simulink model "lab3_buck_closed_loop"  (R2025b)
settings: Solver=VariableStepAuto  StartTime=0.0  StopTime=2  RelTol=1e-3
settings Model: Creator=Fer Alexandru  LastModifiedBy=Fer Alexandru

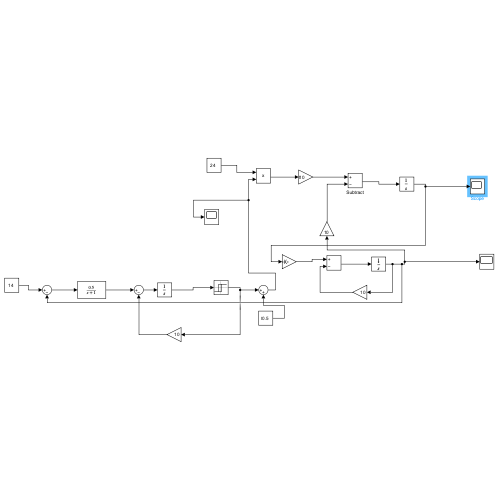
[thumbnail: Simulink's stored preview of the top-level diagram]
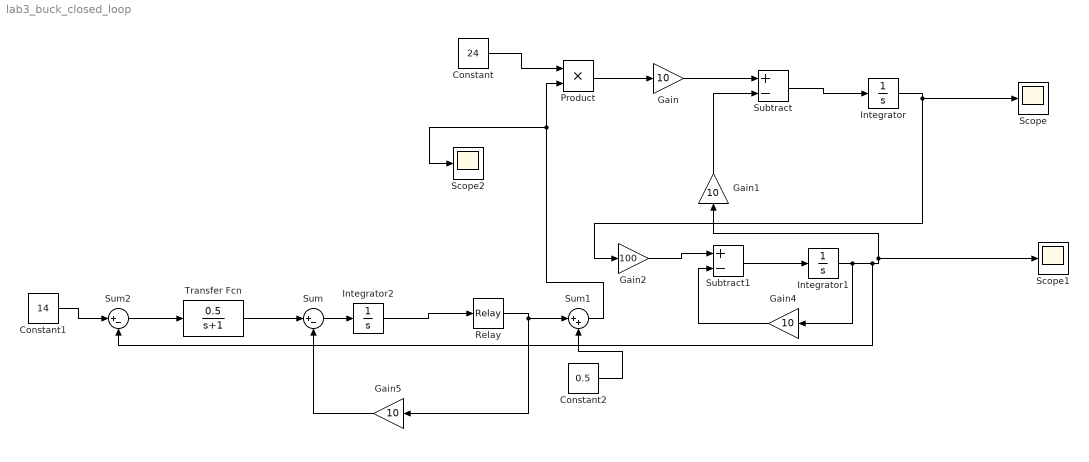
== system lab3_buck_closed_loop ==
  Constant : Constant  Value=24
  Constant1 : Constant  Value=14
  Constant2 : Constant  Value=0.5
  Gain{,1,4..5} (4 alike) : Gain  Gain=10
  Gain2 : Gain  Gain=100
  Integrator : Integrator
  Integrator1 : Integrator
  Integrator2 : Integrator
  Product : Product
  Relay : Relay  OnSwitchValue=0.01  OffSwitchValue=-0.01  OnOutputValue=0.5  OffOutputValue=-0.5
  Scope : Scope
      settings: ActiveDisplayYMinimum=-1.5329376515278401  ActiveDisplayYMaximum=5.42603829532149
  Scope1 : Scope
      settings: ActiveDisplayYMinimum=-0.95807079754853852  ActiveDisplayYMaximum=21.033846575975481
  Scope2 : Scope
      settings: ActiveDisplayYMinimum=0.69234035326086962  ActiveDisplayYMaximum=0.71187160326086951  DataLoggingVariableName=ScopeData2
  Subtract : Sum  Inputs=+-
  Subtract1 : Sum  Inputs=+-
  Sum : Sum  Inputs=|+-
  Sum1 : Sum  Inputs=|++
  Sum2 : Sum  Inputs=|+-
  Transfer Fcn : TransferFcn  Numerator=[0.5]  Denominator=[1 1]
  wires:
  Constant/1 -> Product/1
  Product/1 -> Gain/1
  Gain/1 -> Subtract/1
  Subtract/1 -> Integrator/1
  Gain1/1 -> Subtract/2
  Integrator/1 -> Scope/1, Gain2/1
  Gain2/1 -> Subtract1/1
  Subtract1/1 -> Integrator1/1
  Gain4/1 -> Subtract1/2
  Integrator1/1 -> Gain4/1, Sum2/2, Scope1/1, Gain1/1
  Relay/1 -> Sum1/1, Gain5/1
  Gain5/1 -> Sum/2
  Sum/1 -> Integrator2/1
  Integrator2/1 -> Relay/1
  Transfer Fcn/1 -> Sum/1
  Constant2/1 -> Sum1/2
  Sum1/1 -> Scope2/1, Product/2
  Sum2/1 -> Transfer Fcn/1
  Constant1/1 -> Sum2/1
